simulink model "prelab6"  (R2021a)
settings: Solver=VariableStepAuto  StartTime=0.0  StopTime=0.005  MaxStep=1e-6  RelTol=1e-6
libraries: dsparch4 x2, dspsigops x1
settings Model: Creator=Mataya  LastModifiedBy=Mataya

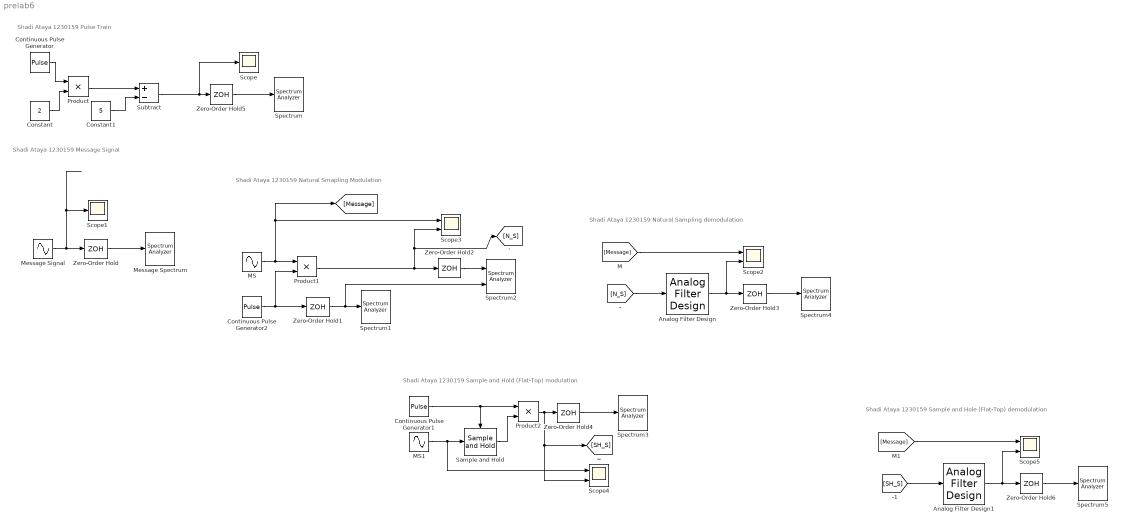
== system prelab6 ==
  note: Shadi Ataya 1230159
      | Sample and Hold (Flat-Top) modulation
  note: Shadi Ataya 1230159
      | Natural Sampling demodulation
  note: Shadi Ataya 1230159
      | Natural Smapling Modulation
  note: Shadi Ataya 1230159
      | Pulse Train
  note: Shadi Ataya 1230159
      | Message Signal
  note: Shadi Ataya 1230159
      | Sample and Hole (Flat-Top) demodulation
  Analog Filter Design : dsparch4/Analog Filter Design  method=Butterworth  filttype=Lowpass  N=6  Wlo=3500*pi*2  Whi=80  Rp=2  Rs=40
  Analog Filter Design1 : dsparch4/Analog Filter Design  method=Butterworth  filttype=Lowpass  N=4  Wlo=3500*pi*2  Whi=80  Rp=2  Rs=40
  Constant : Constant  Value=2
  Constant1 : Constant  Value=5
  Continuous Pulse Generator : DiscretePulseGenerator  PulseType=Time based  Amplitude=5  Period=0.001  PulseWidth=50
  Continuous Pulse Generator1 : DiscretePulseGenerator  PulseType=Time based  Period=6.667e-5  PulseWidth=50
  Continuous Pulse Generator2 : DiscretePulseGenerator  PulseType=Time based  Period=6.667e-5  PulseWidth=50
  MS : Sin  Amplitude=5  Frequency=3000*2*pi  Phase=pi/2  SampleTime=0
  MS1 : Sin  Amplitude=5  Frequency=3000*2*pi  Phase=pi/2  SampleTime=0
  Message Spectrum : SpectrumAnalyzer
  Message Signal : Sin  Frequency=500*2*pi  Phase=pi/2  SampleTime=0
  Product : Product
  Product1 : Product
  Product2 : Product
  Sample and Hold : dspsigops/Sample and Hold  trig=Rising edge  initCond=0  latchinput=off
  Scope : Scope
  Scope1 : Scope
  Scope{2..5} (4 alike) : Scope  NumInputPorts=2
  "Spectrum " : SpectrumAnalyzer
  Spectrum{1,3..5} (4 alike) : SpectrumAnalyzer
  Spectrum2 : SpectrumAnalyzer  NumInputPorts=2
  Subtract : Sum  Inputs=+-
  Zero-Order Hold : ZeroOrderHold  SampleTime=1/10000
  Zero-Order Hold1 : ZeroOrderHold  SampleTime=1/50000
  Zero-Order Hold2 : ZeroOrderHold  SampleTime=1/50000
  Zero-Order Hold3 : ZeroOrderHold  SampleTime=1/20000
  Zero-Order Hold4 : ZeroOrderHold  SampleTime=1/50000
  Zero-Order Hold5 : ZeroOrderHold  SampleTime=1/10000
  Zero-Order Hold6 : ZeroOrderHold  SampleTime=1/20000
  wires:
  Constant1/1 -> Subtract/2
  Constant/1 -> Product/2
  Product/1 -> Subtract/1
  Zero-Order Hold5/1 -> "Spectrum "/1
  Subtract/1 -> Zero-Order Hold5/1, Scope/1
  Continuous Pulse Generator/1 -> Product/1
  Zero-Order Hold/1 -> Message Spectrum/1
  Message Signal/1 -> Zero-Order Hold/1, Scope1/1
  MS/1 -> Product1/1, [Message], Scope3/1
  Zero-Order Hold2/1 -> Spectrum2/1
  Product1/1 -> Scope3/2, [N_S], Zero-Order Hold2/1
  Continuous Pulse Generator2/1 -> Zero-Order Hold1/1, Product1/2
  Zero-Order Hold1/1 -> Spectrum2/2, Spectrum1/1
  Analog Filter Design/1 -> Zero-Order Hold3/1, Scope2/2
  Zero-Order Hold3/1 -> Spectrum4/1
  [Message] -> Scope2/1
  [N_S] -> Analog Filter Design/1
  Sample and Hold/1 -> Product2/2
  MS1/1 -> Scope4/1, Sample and Hold/1
  Continuous Pulse Generator1/1 -> Sample and Hold/Trigger, Product2/1
  Product2/1 -> Scope4/2, [SH_S], Zero-Order Hold4/1
  Zero-Order Hold4/1 -> Spectrum3/1
  Analog Filter Design1/1 -> Zero-Order Hold6/1, Scope5/2
  [Message] -> Scope5/1
  Zero-Order Hold6/1 -> Spectrum5/1
  [SH_S] -> Analog Filter Design1/1
